simulink model "pioneerSNL"  (R2023b)
settings: Solver=ode23t  StartTime=0  StopTime=1300  FixedStep=0.05  MaxStep=0.05  RelTol=1e-3
values from neighbouring files (symbols this model uses):
  aboveWaterMass = 0    [wecSimInputFile.m]
  L0 = 15+19.8    (= 34.8)    [buildMCR.m]    (also in wecSimInputFile.m)
  polyNom = 1.0e+04*[1.9488   -0.0390   -1.3588    0.8094   -0.0004]    [wecSimInputFile.m]
  simu = simulationClass()    [wecSimInputFile.m]
  waves = waveClass('spectrumImportFullDir')    [wecSimInputFile.m]
undefined symbols (not defined in the file or in its folder): body, cable, constraint, geometry, hydroData, pto, X, Y, Z
libraries: nesl_utility x21, sm_lib x17, WECSim_Lib_Body_Elements x7, WECSim_Lib_PTOs x3, WECSim_Lib_Constraints x2, WECSim_Lib_Cables x1, WECSim_Lib_Moorings x1, WECSim_Lib_Frames x1
(part 2 of 2)

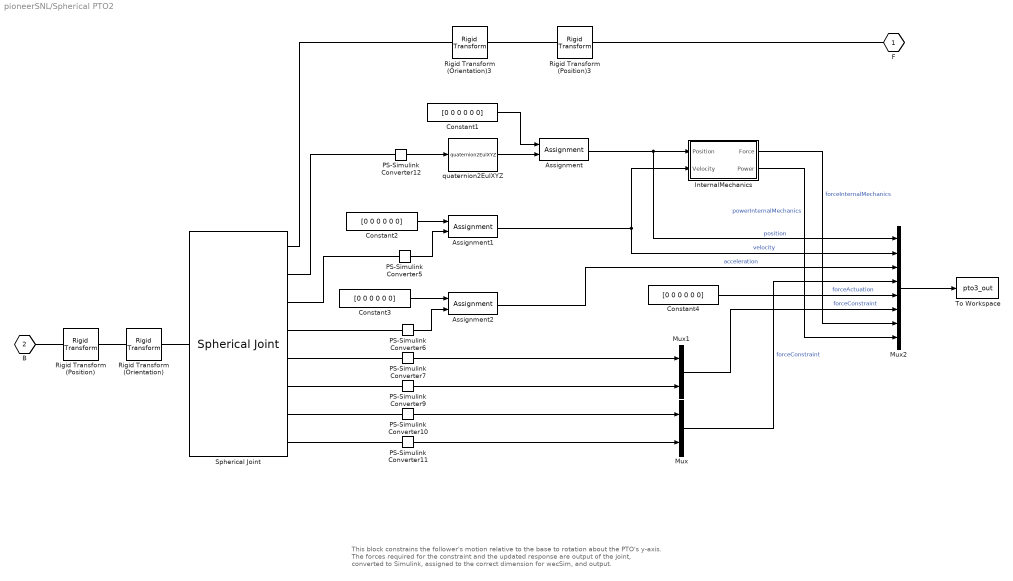
== system pioneerSNL/Spherical PTO2 ==
  note: This block constrains the follower's motion relative to the base to rotation about the PTO's y-axis. The forces required for the constraint and the updated response are output of the joint, converted to Simulink, assigned to the correct dimension for wecSim, and output.
  Assignment : Assignment  IndexOptions=Index vector (dialog)  Indices=[4 5 6]  OutputSizes=1
  Assignment1 : Assignment  IndexOptions=Index vector (dialog)  Indices=[4 5 6]  OutputSizes=1
  Assignment2 : Assignment  IndexOptions=Index vector (dialog)  Indices=[4,5,6]  OutputSizes=1
  Constant{1..4} (4 alike) : Constant  Value=[0 0 0 0 0 0]
  InternalMechanics : Subsystem
  Mux : Mux  Inputs=2
  Mux1 : Mux  Inputs=2
  Mux2 : Mux  Inputs=8
  PS-Simulink Converter{5..7,9..12} (7 alike) : nesl_utility/PS-Simulink Converter  PhysicalDomain=network_engine_domain  SubClassName=ps_output  LeftPortType=input  RightPortType=output  PseudoPeriodic=off  Frequencies=[]  VectorFormat=1-D array  Unit=inherit  AffineConversion=off
  Rigid Transform (Orientation) : sm_lib/Frames and Transforms/Rigid Transform  TranslationMethod=None  TranslationStandardOffset=0  TranslationStandardOffsetUnits=m  TranslationStandardAxis=+Z  TranslationCartesianOffset=constraint.initial.displacement+constraint.location  TranslationCartesianOffsetUnits=m  TranslationROffset=0  TranslationROffsetUnits=m  TranslationZOffset=0  TranslationZOffsetUnits=m  TranslationThetaOffset=0  TranslationThetaOffsetUnits=deg  RotationMethod=RotationMatrix  RotationAngleUnits=deg  RotationStandardAxis=+Z  RotationAngle=0.0  RotationArbitraryAxis=[0 0 1]  FollAlignAxisA=+X  BaseAlignAxisA=+Y  FollAlignAxisB=+Y  BaseAlignAxisB=+Z  RotationSequenceAxes=FollowerAxes  RotationSequence=XYX  RotationSequenceAngles=[0 0 0]  RotationSequenceAnglesUnits=deg  RotationMatrix=pto.orientation.rotationMatrix  Quaternion=[1 0 0 0]
  Rigid Transform (Orientation)3 : sm_lib/Frames and Transforms/Rigid Transform  TranslationMethod=None  TranslationStandardOffset=0  TranslationStandardOffsetUnits=m  TranslationStandardAxis=+Z  TranslationCartesianOffset=constraint.initial.displacement+constraint.location  TranslationCartesianOffsetUnits=m  TranslationROffset=0  TranslationROffsetUnits=m  TranslationZOffset=0  TranslationZOffsetUnits=m  TranslationThetaOffset=0  TranslationThetaOffsetUnits=deg  RotationMethod=RotationMatrix  RotationAngleUnits=deg  RotationStandardAxis=+Z  RotationAngle=0.0  RotationArbitraryAxis=[0 0 1]  FollAlignAxisA=+X  BaseAlignAxisA=+Y  FollAlignAxisB=+Y  BaseAlignAxisB=+Z  RotationSequenceAxes=FollowerAxes  RotationSequence=XYX  RotationSequenceAngles=[0 0 0]  RotationSequenceAnglesUnits=deg  RotationMatrix=pto.orientation.rotationMatrix  Quaternion=[1 0 0 0]
  Rigid Transform (Position) : sm_lib/Frames and Transforms/Rigid Transform  TranslationMethod=Cartesian  TranslationStandardOffset=0  TranslationStandardOffsetUnits=m  TranslationStandardAxis=+Z  TranslationCartesianOffset=pto.initial.displacement+pto.location  TranslationCartesianOffsetUnits=m  TranslationROffset=0  TranslationROffsetUnits=m  TranslationZOffset=0  TranslationZOffsetUnits=m  TranslationThetaOffset=0  TranslationThetaOffsetUnits=deg  RotationMethod=None  RotationAngleUnits=deg  RotationStandardAxis=+Z  RotationAngle=0.0  RotationArbitraryAxis=[0 0 1]  FollAlignAxisA=+X  BaseAlignAxisA=+Y  FollAlignAxisB=+Y  BaseAlignAxisB=+Z  RotationSequenceAxes=FollowerAxes  RotationSequence=XYX  RotationSequenceAngles=[0 0 0]  RotationSequenceAnglesUnits=deg  RotationMatrix=[1 0 0; 0 1 0; 0 0 1]  Quaternion=[1 0 0 0]
  Rigid Transform (Position)3 : sm_lib/Frames and Transforms/Rigid Transform  TranslationMethod=Cartesian  TranslationStandardOffset=0  TranslationStandardOffsetUnits=m  TranslationStandardAxis=+Z  TranslationCartesianOffset=pto.initial.displacement+pto.location  TranslationCartesianOffsetUnits=m  TranslationROffset=0  TranslationROffsetUnits=m  TranslationZOffset=0  TranslationZOffsetUnits=m  TranslationThetaOffset=0  TranslationThetaOffsetUnits=deg  RotationMethod=None  RotationAngleUnits=deg  RotationStandardAxis=+Z  RotationAngle=0.0  RotationArbitraryAxis=[0 0 1]  FollAlignAxisA=+X  BaseAlignAxisA=+Y  FollAlignAxisB=+Y  BaseAlignAxisB=+Z  RotationSequenceAxes=FollowerAxes  RotationSequence=XYX  RotationSequenceAngles=[0 0 0]  RotationSequenceAnglesUnits=deg  RotationMatrix=[1 0 0; 0 1 0; 0 0 1]  Quaternion=[1 0 0 0]
  Spherical Joint : sm_lib/Joints/Spherical Joint  JointMode=Normal  SenseConstraintForce=on  SenseConstraintForceX=off  SenseConstraintForceY=off  SenseConstraintForceZ=off  SenseConstraintTorque=on  SenseConstraintTorqueX=off  SenseConstraintTorqueY=off  SenseConstraintTorqueZ=off  SenseTotalForce=on  SenseTotalForceX=off  SenseTotalForceY=off  SenseTotalForceZ=off  SenseTotalTorque=on  SenseTotalTorqueX=off  SenseTotalTorqueY=off  SenseTotalTorqueZ=off  CompositeWrenchDir=BaseOnFollower  CompositeWrenchFrame=BaseFrame  EqPosRotationMethod=None  EqPosRotationAngleUnits=deg  EqPosRotationStandardAxis=+Z  EqPosRotationAngle=0.0  EqPosRotationArbitraryAxis=[0 0 1]  EqPosFollAlignAxisA=+X  EqPosBaseAlignAxisA=+Y  EqPosFollAlignAxisB=+Y  EqPosBaseAlignAxisB=+Z  EqPosRotationSequenceAxes=FollowerAxes  EqPosRotationSequence=XYX  EqPosRotationSequenceAngles=[0 0 0]  EqPosRotationSequenceAnglesUnits=deg  EqPosRotationMatrix=[1 0 0; 0 1 0; 0 0 1]  EqPosQuaternion=[1 0 0 0]  SpringStiffness=pto.stiffness  SpringStiffnessUnits=N*m/rad  DampingCoefficient=pto.damping  DampingCoefficientUnits=N*m/(rad/s)  ActuateTorqueX=off  ActuateTorqueY=off  ActuateTorqueZ=off  ActuateTorque=off  TorqueActuationMode=NoTorque  MotionActuationMode=ComputedMotion  ActuationFrame=BaseFrame  SensePosition=on  SenseVelocityX=off  SenseVelocityY=off  SenseVelocityZ=off  SenseVelocity=on  SenseAccelerationX=off  SenseAccelerationY=off  SenseAccelerationZ=off  SenseAcceleration=on  SenseTorqueX=off  SenseTorqueY=off  SenseTorqueZ=off  SenseTorqueForce=off  SenseLowerLimitTorqueMag=off  SenseUpperLimitTorqueMag=off  SensingFrame=BaseFrame  LowerLimitSpecify=off  LowerLimitBound=15  LowerLimitBoundUnits=deg  LowerLimitStiffness=1e4  LowerLimitStiffnessUnits=N*m/deg  LowerLimitDamping=10  LowerLimitDampingUnits=N*m/(deg/s)  LowerLimitTransitionRegionWidth=0.1  LowerLimitTransitionRegionWidthUnits=deg  UpperLimitSpecify=off  UpperLimitBound=45  UpperLimitBoundUnits=deg  UpperLimitStiffness=1e4  UpperLimitStiffnessUnits=N*m/deg  UpperLimitDamping=10  UpperLimitDampingUnits=N*m/(deg/s)  UpperLimitTransitionRegionWidth=0.1  UpperLimitTransitionRegionWidthUnits=deg  PositionTargetRotationMethod=None  PositionTargetRotationAngleUnits=deg  PositionTargetRotationStandardAxis=+Z  PositionTargetRotationAngle=0.0  PositionTargetRotationArbitraryAxis=[0 0 1]  PositionTargetFollAlignAxisA=+X  PositionTargetBaseAlignAxisA=+Y  PositionTargetFollAlignAxisB=+Y  PositionTargetBaseAlignAxisB=+Z  PositionTargetRotationSequenceAxes=FollowerAxes  PositionTargetRotationSequence=XYX  PositionTargetRotationSequenceAngles=[0 0 0]  PositionTargetRotationSequenceAnglesUnits=deg  PositionTargetRotationMatrix=[1 0 0; 0 1 0; 0 0 1]  PositionTargetQuaternion=[1 0 0 0]  PositionTargetSpecify=off  PositionTargetPriority=High  VelocityTargetValue=[0 0 0]  VelocityTargetValueUnits=deg/s  VelocityTargetSpecify=off  VelocityTargetPriority=High  VelocityTargetInFollowerFrame=on
  To Workspace : ToWorkspace  VariableName=pto3_out  SaveFormat=Structure With Time  SampleTime=simu.dtOut
  quaternion2EulXYZ : WECSim_Lib_Body_Elements/Rigid Body/Hydrodynamic Body/Structure/Motion Sensor/quaternion2EulXYZ  SystemSampleTime=-1  VariantActivationTime=update diagram  AllowFlexibleInterface=on  Latency=0  AutoFrameSizeCalculation=off
  F : PMIOPort  Side=Right
  B : PMIOPort  Port=2  Side=Left
  wires:
  Mux/1 -> Mux2/4  "forceConstraint"
  Assignment2/1 -> Mux2/3  "acceleration"
  PS-Simulink Converter11/1 -> Mux/2
  PS-Simulink Converter12/1 -> quaternion2EulXYZ/1
  Constant3/1 -> Assignment2/1
  InternalMechanics/2(Power) -> Mux2/8  "powerInternalMechanics"
  Assignment1/1 -> Mux2/2, InternalMechanics/2(Velocity)  "velocity"
  Constant2/1 -> Assignment1/1
  Constant4/1 -> Mux2/5  "forceActuation"
  PS-Simulink Converter6/1 -> Assignment2/2
  Assignment/1 -> Mux2/1, InternalMechanics/1(Position)  "position"
  PS-Simulink Converter7/1 -> Mux1/1
  PS-Simulink Converter10/1 -> Mux/1
  PS-Simulink Converter5/1 -> Assignment1/2
  PS-Simulink Converter9/1 -> Mux1/2
  quaternion2EulXYZ/1 -> Assignment/2
  Constant1/1 -> Assignment/1
  Mux2/1 -> To Workspace/1
  InternalMechanics/1(Force) -> Mux2/7  "forceInternalMechanics"
  Mux1/1 -> Mux2/6  "forceConstraint"
  connections:
  Rigid Transform (Orientation)/RConn1 -- Spherical Joint/LConn1
  Spherical Joint/RConn8 -- PS-Simulink Converter11/LConn1
  Spherical Joint/RConn2 -- PS-Simulink Converter12/LConn1
  Spherical Joint/RConn7 -- PS-Simulink Converter10/LConn1
  Rigid Transform (Orientation)3/LConn1 -- Rigid Transform (Position)3/RConn1
  Rigid Transform (Position)/LConn1 -- B/RConn1
  Spherical Joint/RConn4 -- PS-Simulink Converter6/LConn1
  Spherical Joint/RConn5 -- PS-Simulink Converter7/LConn1
  Spherical Joint/RConn1 -- Rigid Transform (Orientation)3/RConn1
  Rigid Transform (Orientation)/LConn1 -- Rigid Transform (Position)/RConn1
  Spherical Joint/RConn6 -- PS-Simulink Converter9/LConn1
  Rigid Transform (Position)3/LConn1 -- F/RConn1
  Spherical Joint/RConn3 -- PS-Simulink Converter5/LConn1

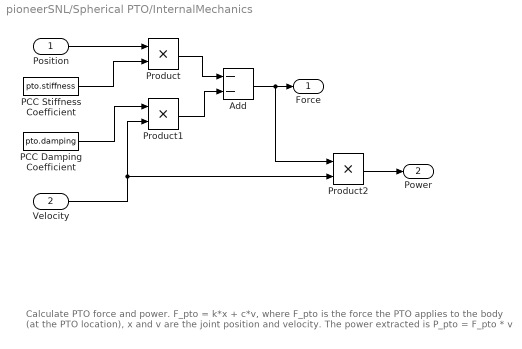
== system pioneerSNL/Spherical PTO/InternalMechanics ==
  note: Calculate PTO force and power.
      |
      | F_pto  = k*x + c*v,
      | where F_pto is the force the PTO applies to the body (at the PTO location), x and v are the joint position and velocity.
      |
      | The power extracted is
      | P_pto = F_pto * v
  Position : Inport
  Velocity : Inport  Port=2
  Add : Sum  Inputs=--
  PCC Damping Coefficient : Constant  Value=pto.damping
  PCC Stiffness Coefficient : Constant  Value=pto.stiffness
  Product : Product  Inputs=**
  Product1 : Product  Inputs=**
  Product2 : Product  Inputs=**
  Force : Outport
  Power : Outport  Port=2
  wires:
  Product1/1 -> Add/2
  Product/1 -> Add/1
  Velocity/1 -> Product1/2, Product2/2
  Add/1 -> Force/1, Product2/1
  Position/1 -> Product/1
  PCC Stiffness Coefficient/1 -> Product/2
  Product2/1 -> Power/1
  PCC Damping Coefficient/1 -> Product1/1

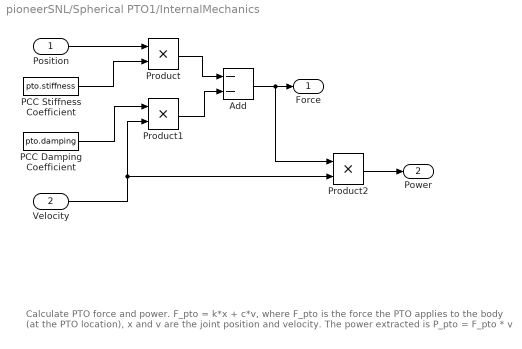
== system pioneerSNL/Spherical PTO1/InternalMechanics ==
  note: Calculate PTO force and power.
      |
      | F_pto  = k*x + c*v,
      | where F_pto is the force the PTO applies to the body (at the PTO location), x and v are the joint position and velocity.
      |
      | The power extracted is
      | P_pto = F_pto * v
  Position : Inport
  Velocity : Inport  Port=2
  Add : Sum  Inputs=--
  PCC Damping Coefficient : Constant  Value=pto.damping
  PCC Stiffness Coefficient : Constant  Value=pto.stiffness
  Product : Product  Inputs=**
  Product1 : Product  Inputs=**
  Product2 : Product  Inputs=**
  Force : Outport
  Power : Outport  Port=2
  wires:
  Product1/1 -> Add/2
  Product/1 -> Add/1
  Velocity/1 -> Product1/2, Product2/2
  Add/1 -> Force/1, Product2/1
  Position/1 -> Product/1
  PCC Stiffness Coefficient/1 -> Product/2
  Product2/1 -> Power/1
  PCC Damping Coefficient/1 -> Product1/1

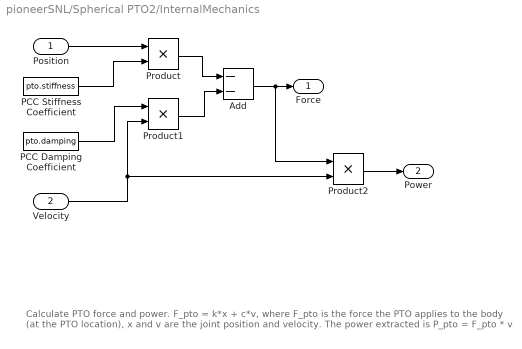
== system pioneerSNL/Spherical PTO2/InternalMechanics ==
  note: Calculate PTO force and power.
      |
      | F_pto  = k*x + c*v,
      | where F_pto is the force the PTO applies to the body (at the PTO location), x and v are the joint position and velocity.
      |
      | The power extracted is
      | P_pto = F_pto * v
  Position : Inport
  Velocity : Inport  Port=2
  Add : Sum  Inputs=--
  PCC Damping Coefficient : Constant  Value=pto.damping
  PCC Stiffness Coefficient : Constant  Value=pto.stiffness
  Product : Product  Inputs=**
  Product1 : Product  Inputs=**
  Product2 : Product  Inputs=**
  Force : Outport
  Power : Outport  Port=2
  wires:
  Product1/1 -> Add/2
  Product/1 -> Add/1
  Velocity/1 -> Product1/2, Product2/2
  Add/1 -> Force/1, Product2/1
  Position/1 -> Product/1
  PCC Stiffness Coefficient/1 -> Product/2
  Product2/1 -> Power/1
  PCC Damping Coefficient/1 -> Product1/1

== matlab function pioneerSNL/CustomMooring/MATLAB Function ==
  data: displacement input; Tension output; polyNom parameter; L0 parameter
function Tension = fcn(displacement,polyNom,L0)

% initialize output
Tension = 0;

% calculate according to input file polynomial and unstretched length
strain = (displacement-L0)/L0;
arg = max([strain;0]);
Tension = polyval(polyNom,arg);

end
